simulink model "EKFSim"  (R2025b)
settings: Solver=FixedStepAuto  StartTime=0.0  StopTime=4500  RelTol=1e-3
values from neighbouring files (symbols this model uses):
  C1_bp = interp1(ECM.SOC_table, ECM.C1_table, SOC_bp, 'pchip')    [preparer_LUT_pour_EKFSim.m]
  OCV_bp = ppval(ECM.pp_OCV, SOC_bp)    [preparer_LUT_pour_EKFSim.m]
  R0_bp = interp1(ECM.SOC_table, ECM.R0_table, SOC_bp, 'pchip')    [preparer_LUT_pour_EKFSim.m]
  R1_bp = interp1(ECM.SOC_table, ECM.R1_table, SOC_bp, 'pchip')    [preparer_LUT_pour_EKFSim.m]
  SOC_bp = (5:1:100)' / 100    [preparer_LUT_pour_EKFSim.m]
libraries: fl_lib x7, nesl_utility x7
settings Model: Creator=WL  LastModifiedBy=SAT
settings SolverCC: AlgebraicLoopSolver=TrustRegion
settings DataIOCC: ReturnWorkspaceOutputs=off
settings DebuggingCC: UnconnectedInputMsg=warning  UnconnectedOutputMsg=warning  UnconnectedLineMsg=warning  ArithmeticOperatorsInVariantConditions=warning
settings ModelReferenceCC: EnableRefExpFcnMdlSchedulingChecks=on
settings SFSimCC: SimUseLocalCustomCode=off  CustomCodeUndefinedFunction=UseInterfaceOnly
settings RTWCC: GenCodeOnly=on  RTWUseLocalCustomCode=off  GPUComputeCapability=3.5
settings CodeAppCC: StateflowObjectComments=on

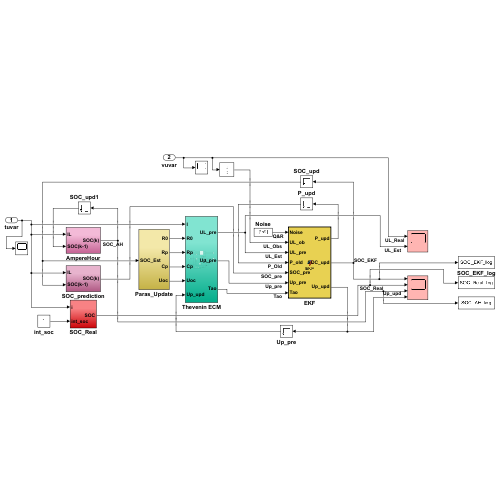
[thumbnail: Simulink's stored preview of the top-level diagram]
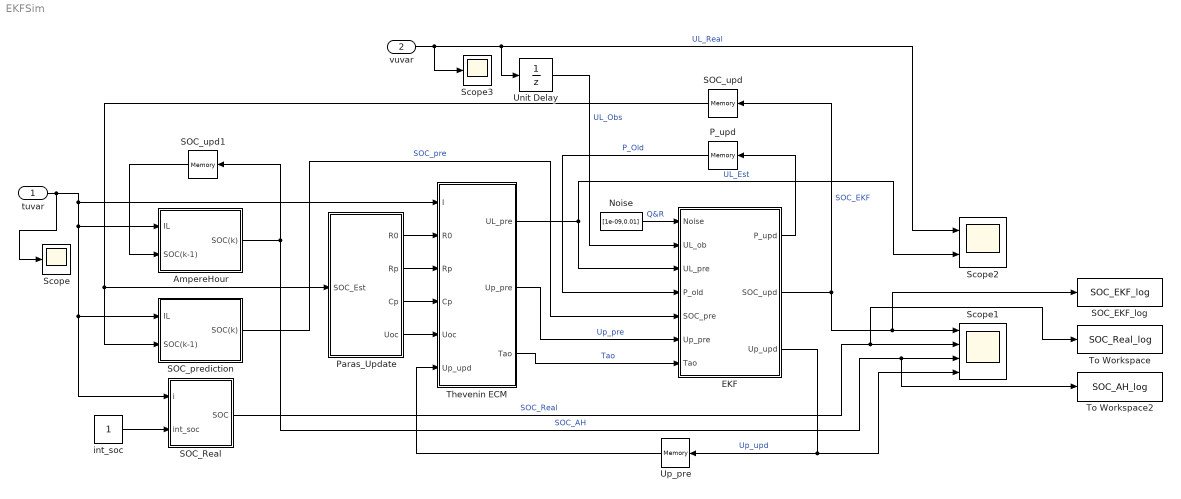
== system EKFSim ==
  tuvar : Inport  OutDataTypeStr=double
  vuvar : Inport  Port=2  OutDataTypeStr=double
  AmpereHour : Subsystem
  EKF : MATLAB Function  TreatAsAtomicUnit=on
  Noise : Constant  Value=[1e-09,0.01]
  P_upd : Memory  InitialCondition=[0.02 0 0 0.01]  InheritSampleTime=on  LinearizeAsDelay=on
  Paras_Update : Subsystem
  SOC_EKF_log : ToWorkspace  VariableName=SOC_EKF_log  SampleTime=-1
  SOC_Real : Subsystem
  SOC_prediction : Subsystem
  SOC_upd : Memory  InitialCondition=1  InheritSampleTime=on  LinearizeAsDelay=on
  SOC_upd1 : Memory  InitialCondition=1  InheritSampleTime=on  LinearizeAsDelay=on
  Scope : Scope
      settings: ActiveDisplayYMinimum=-18.981393680658311  ActiveDisplayYMaximum=11.78942945455692
  Scope1 : Scope  NumInputPorts=4
      settings: ActiveDisplayYMinimum=-0.2544970250554105  ActiveDisplayYMaximum=1.3066318096988883  DataLoggingVariableName=ScopeData2
  Scope2 : Scope  NumInputPorts=2
      settings: ActiveDisplayYMinimum=2.9853  ActiveDisplayYMaximum=4.38231  DataLoggingVariableName=ScopeData2
  Scope3 : Scope
      settings: ActiveDisplayYMinimum=-13.743145742790805  ActiveDisplayYMaximum=10.36659934742335  DataLoggingVariableName=ScopeData3
  Thevenin ECM : Subsystem
  To Workspace : ToWorkspace  VariableName=SOC_Real_log  SampleTime=-1
  To Workspace2 : ToWorkspace  VariableName=SOC_AH_log  SampleTime=-1
  Unit Delay : UnitDelay  InitialCondition=4.107  SampleTime=0.1  HasFrameUpgradeWarning=on
  Up_pre : Memory  InheritSampleTime=on  LinearizeAsDelay=on
  int_soc : Constant
  wires:
  Paras_Update/4(Uoc) -> Thevenin ECM/5(Uoc)
  Paras_Update/1(R0) -> Thevenin ECM/2(R0)
  int_soc/1 -> SOC_Real/2(int_soc)
  Paras_Update/3(Cp) -> Thevenin ECM/4(Cp)
  Paras_Update/2(Rp) -> Thevenin ECM/3(Rp)
  Thevenin ECM/1(UL_pre) -> Scope2/2, EKF/3(UL_pre)  "UL_Est"
  vuvar/1 -> Scope3/1, Unit Delay/1, Scope2/1  "UL_Real"
  SOC_Real/1(SOC) -> To Workspace/1, Scope1/2  "SOC_Real"
  Thevenin ECM/2(Up_pre) -> EKF/6(Up_pre)  "Up_pre"
  Noise/1 -> EKF/1(Noise)  "Q&R"
  SOC_prediction/1(SOC(k)) -> EKF/5(SOC_pre)  "SOC_pre"
  P_upd/1 -> EKF/4(P_old)  "P_Old"
  SOC_upd/1 -> SOC_prediction/2(SOC(k-1)), Paras_Update/1(SOC_Est)
  EKF/1(P_upd) -> P_upd/1
  Thevenin ECM/3(Tao) -> EKF/7(Tao)  "Tao"
  EKF/3(Up_upd) -> Scope1/4, Up_pre/1  "Up_upd"
  Up_pre/1 -> Thevenin ECM/6(Up_upd)
  EKF/2(SOC_upd) -> SOC_EKF_log/1, Scope1/1, SOC_upd/1  "SOC_EKF"
  Unit Delay/1 -> EKF/2(UL_ob)  "UL_Obs"
  AmpereHour/1(SOC(k)) -> To Workspace2/1, Scope1/3, SOC_upd1/1  "SOC_AH"
  tuvar/1 -> Scope/1, SOC_prediction/1(IL), SOC_Real/1(i), AmpereHour/1(IL), Thevenin ECM/1(I)
  SOC_upd1/1 -> AmpereHour/2(SOC(k-1))

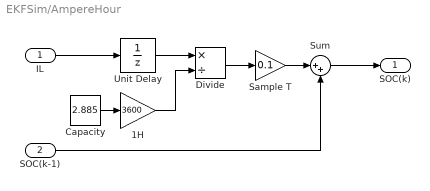
== system EKFSim/AmpereHour ==
  IL : Inport
  SOC(k-1) : Inport  Port=2
  1H : Gain  Gain=3600
  Capacity : Constant  Value=2.885
  Divide : Product  Inputs=*/
  Sample T : Gain  Gain=0.1
  Sum : Sum  Inputs=|++
  Unit Delay : UnitDelay  SampleTime=-1  HasFrameUpgradeWarning=on
  SOC(k) : Outport  VectorParamsAs1DForOutWhenUnconnected=off
  wires:
  Sample T/1 -> Sum/1
  Unit Delay/1 -> Divide/1
  SOC(k-1)/1 -> Sum/2
  IL/1 -> Unit Delay/1
  Sum/1 -> SOC(k)/1
  Capacity/1 -> 1H/1
  1H/1 -> Divide/2
  Divide/1 -> Sample T/1

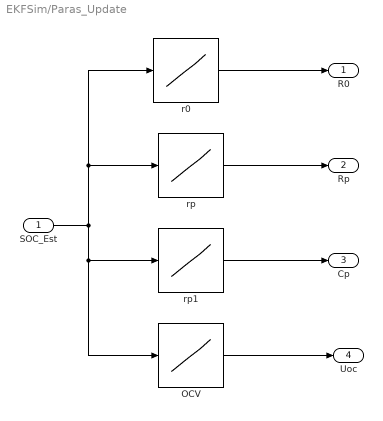
== system EKFSim/Paras_Update ==
  SOC_Est : Inport
  OCV : Lookup_n-D  NumberOfTableDimensions=1  BreakpointsForDimension1=SOC_bp  Table=OCV_bp  ExtrapMethod=Clip  InternalRulePriority=Speed  RndMeth=Simplest
  r0 : Lookup_n-D  NumberOfTableDimensions=1  BreakpointsForDimension1=SOC_bp  Table=R0_bp  ExtrapMethod=Clip  InternalRulePriority=Speed  RndMeth=Simplest
  rp : Lookup_n-D  NumberOfTableDimensions=1  BreakpointsForDimension1=SOC_bp  Table=R1_bp  ExtrapMethod=Clip  InternalRulePriority=Speed  RndMeth=Simplest
  rp1 : Lookup_n-D  NumberOfTableDimensions=1  BreakpointsForDimension1=SOC_bp  Table=C1_bp  ExtrapMethod=Clip  InternalRulePriority=Speed  RndMeth=Simplest
  R0 : Outport  VectorParamsAs1DForOutWhenUnconnected=off
  Rp : Outport  Port=2  VectorParamsAs1DForOutWhenUnconnected=off
  Cp : Outport  Port=3  VectorParamsAs1DForOutWhenUnconnected=off
  Uoc : Outport  Port=4  VectorParamsAs1DForOutWhenUnconnected=off
  wires:
  SOC_Est/1 -> OCV/1, rp1/1, rp/1, r0/1
  rp/1 -> Rp/1
  OCV/1 -> Uoc/1
  r0/1 -> R0/1
  rp1/1 -> Cp/1

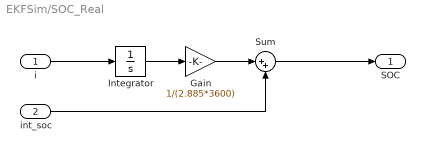
== system EKFSim/SOC_Real ==
  i : Inport
  int_soc : Inport  Port=2
  Gain : Gain  Gain=1/(2.885*3600)
  Integrator : Integrator
  Sum : Sum  Inputs=|++
  SOC : Outport  VectorParamsAs1DForOutWhenUnconnected=off
  wires:
  Gain/1 -> Sum/1
  Integrator/1 -> Gain/1
  int_soc/1 -> Sum/2
  i/1 -> Integrator/1
  Sum/1 -> SOC/1

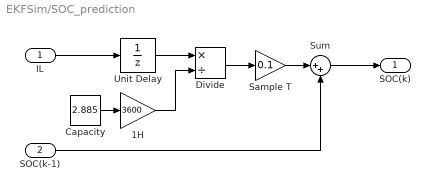
== system EKFSim/SOC_prediction ==
  IL : Inport
  SOC(k-1) : Inport  Port=2
  1H : Gain  Gain=3600
  Capacity : Constant  Value=2.885
  Divide : Product  Inputs=*/
  Sample T : Gain  Gain=0.1
  Sum : Sum  Inputs=|++
  Unit Delay : UnitDelay  SampleTime=-1  HasFrameUpgradeWarning=on
  SOC(k) : Outport  VectorParamsAs1DForOutWhenUnconnected=off
  wires:
  Sample T/1 -> Sum/1
  Unit Delay/1 -> Divide/1
  SOC(k-1)/1 -> Sum/2
  IL/1 -> Unit Delay/1
  Sum/1 -> SOC(k)/1
  Capacity/1 -> 1H/1
  1H/1 -> Divide/2
  Divide/1 -> Sample T/1

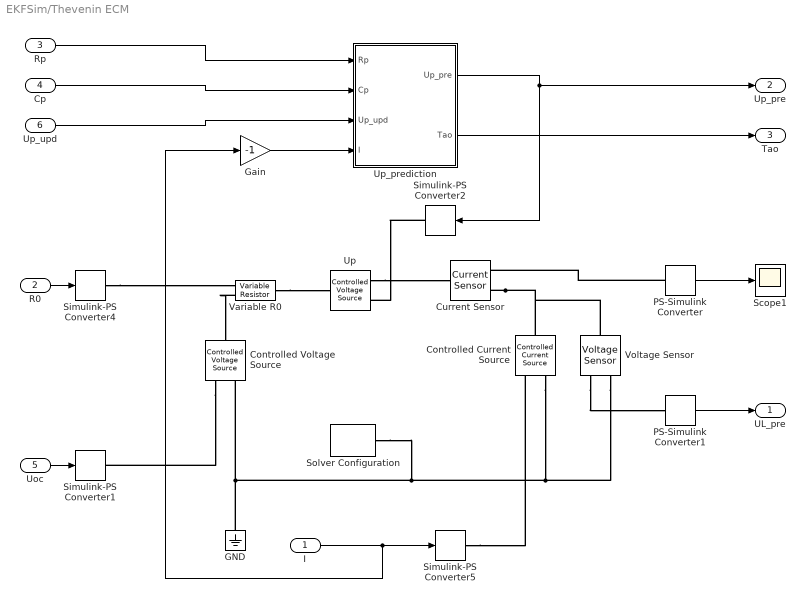
== system EKFSim/Thevenin ECM ==
  I : Inport
  R0 : Inport  Port=2
  Rp : Inport  Port=3
  Cp : Inport  Port=4
  Uoc : Inport  Port=5
  Up_upd : Inport  Port=6
  Controlled Current Source : fl_lib/Electrical/Electrical Sources/Controlled Current Source
  Controlled Voltage Source : fl_lib/Electrical/Electrical Sources/Controlled Voltage Source
  Current Sensor : fl_lib/Electrical/Electrical Sensors/Current Sensor
  GND : fl_lib/Electrical/Electrical Elements/Electrical Reference
  Gain : Gain  Gain=-1
  PS-Simulink Converter : nesl_utility/PS-Simulink Converter  PhysicalDomain=network_engine_domain  SubClassName=ps_output  LeftPortType=input  RightPortType=output  PseudoPeriodic=off  Frequencies=[]  VectorFormat=1-D array  Unit=A  AffineConversion=off
  PS-Simulink Converter1 : nesl_utility/PS-Simulink Converter  PhysicalDomain=network_engine_domain  SubClassName=ps_output  LeftPortType=input  RightPortType=output  PseudoPeriodic=off  Frequencies=[]  VectorFormat=1-D array  Unit=V  AffineConversion=off
  Scope1 : Scope
      settings: ActiveDisplayYMinimum=-63.1775  ActiveDisplayYMaximum=62.5975
  Simulink-PS Converter{1..2,4..5} (4 alike) : nesl_utility/Simulink-PS Converter  PhysicalDomain=network_engine_domain  SubClassName=ps_input  LeftPortType=input  RightPortType=output  PseudoPeriodic=off  Frequencies=[]  NoiseDistribution=none  NoiseParameters=[]  Unit=1  AffineConversion=off  FilteringAndDerivatives=zero  SimscapeFilterOrder=1  InputFilterTimeConstant=0.001  UdotUserProvided=0
  Solver Configuration : nesl_utility/Solver Configuration  PhysicalDomain=network_engine_domain  SubClassName=solver  LeftPortType=input  RightPortType=generic  Tones=[]  Harmonics=[]  SimulateNoise=off  Profile=off  UseLocalSampling=off  EnableSwitchedLinearOptims=on  FrequencyDomain=off  UseCCode=off  RelTol=0.001  AbsTol=1e-06  MinStep=1e-09  ToWorkspace=off  RevertToSquareIcSolve=off  NumHomotopyIterations=100  PhasorMode=off  PhasorModeNumHarmonics=1  ConsistencySolver=NEWTON_FTOL  IndexReductionMethod=DerivativeReplacement  DoDC=off  ResidualTolerance=1e-09  ConsistencyTolSource=GLOBAL  ConsistencyAbsTol=0.001  ConsistencyRelTol=0.001  ConsistencyTolFactor=0.001  UseLocalSolver=off  LocalSolverChoice=NE_BACKWARD_EULER_ADVANCER  ResolveIndetEquations=on  FunctionEvalNumThread=1  LocalSolverSampleTime=0.001  DoFixedCost=off  MaxNonlinIter=3  MaxModeIter=2  ComputeImpulses=off  ImpulseIterations=2  LinearAlgebra=Sparse  LinearAlgebraNumThread=0  EquationFormulation=NE_TIME_EF  DelaysMemoryBudget=1024  AutomaticFiltering=on  FilteringTimeConstant=0.001  PartitionStorageMethod=AS_NEEDED  PartitionMemoryBudget=1024  PartitionMethod=FAST  MultibodyUseLocalSolver=off  MultibodyLocalSolverChoice=ODE1  MultibodyLocalSolverSampleTime=0.001
  Up : fl_lib/Electrical/Electrical Sources/Controlled Voltage Source
  Up_prediction : MATLAB Function  TreatAsAtomicUnit=on
  Variable R0 : fl_lib/Electrical/Electrical Elements/Variable Resistor  Rmin=0 Ohm  thermalEnable=false  thermal_mass=1 J/K  i_specify=off  i_priority=None  i=0 A  i_nominal_specify=off  i_nominal_value=1  i_nominal_unit=A  v_specify=off  v_priority=None  v=0 V  v_nominal_specify=off  v_nominal_value=1  v_nominal_unit=V  T_specify=off  T_priority=None  T=300 K  T_nominal_specify=off  T_nominal_value=1  T_nominal_unit=K
  Voltage Sensor : fl_lib/Electrical/Electrical Sensors/Voltage Sensor
  UL_pre : Outport  VectorParamsAs1DForOutWhenUnconnected=off
  Up_pre : Outport  Port=2  VectorParamsAs1DForOutWhenUnconnected=off
  Tao : Outport  Port=3  VectorParamsAs1DForOutWhenUnconnected=off
  wires:
  PS-Simulink Converter1/1 -> UL_pre/1
  Uoc/1 -> Simulink-PS Converter1/1
  Cp/1 -> Up_prediction/2(Cp)
  Rp/1 -> Up_prediction/1(Rp)
  R0/1 -> Simulink-PS Converter4/1
  I/1 -> Gain/1, Simulink-PS Converter5/1
  PS-Simulink Converter/1 -> Scope1/1
  Up_prediction/1(Up_pre) -> Simulink-PS Converter2/1, Up_pre/1
  Up_upd/1 -> Up_prediction/3(Up_upd)
  Up_prediction/2(Tao) -> Tao/1
  Gain/1 -> Up_prediction/4(I)
  connections:
  Variable R0/LConn2 -- Controlled Voltage Source/LConn1
  Current Sensor/RConn2 -- Voltage Sensor/LConn1 -- Controlled Current Source/LConn1
  Voltage Sensor/RConn2 -- Controlled Current Source/RConn2 -- Solver Configuration/RConn1 -- Controlled Voltage Source/RConn2 -- GND/LConn1
  PS-Simulink Converter/LConn1 -- Current Sensor/RConn1
  Voltage Sensor/RConn1 -- PS-Simulink Converter1/LConn1
  Controlled Voltage Source/RConn1 -- Simulink-PS Converter1/RConn1
  Simulink-PS Converter5/RConn1 -- Controlled Current Source/RConn1
  Simulink-PS Converter4/RConn1 -- Variable R0/LConn1
  Variable R0/RConn1 -- Up/LConn1
  Up/RConn2 -- Current Sensor/LConn1
  Simulink-PS Converter2/RConn1 -- Up/RConn1

== matlab function EKFSim/Thevenin ECM/Up_prediction ==
  data: Rp input; Up_pre output; Cp input; Up_upd input; Tao output; I input
function [Up_pre, Tao] = fcn(Rp, Cp,Up_upd,I)
Ts = 0.1;
Tao = Rp*Cp;
Up_pre = exp(-Ts/Tao)*Up_upd + Rp*(1-exp(-Ts/Tao))*I;
end

== matlab function EKFSim/EKF ==
  data: P_upd output; Noise input; UL_ob input; UL_pre input; P_old input; SOC_pre input; Up_pre input; Tao input; SOC_upd output; Up_upd output
function [P_upd,SOC_upd,Up_upd] = EKF(Noise, UL_ob, UL_pre, P_old, SOC_pre, Up_pre, Tao)
Ts = 0.1;    % <-- MÊME Ts que dans Thevenin ECM
Q = Noise(1);
R = Noise(2);

A1 = 1;
A2 = exp(-Ts/Tao);
A = [A1 0;0 A2];

P_last = [P_old(1) P_old(2);P_old(3) P_old(4)];
P_pre = A*P_last*A' + [Q 0;0 Q];

SOC_vec  = [0.05 0.1 0.15 0.2 0.25 0.3 0.4 0.5 0.6 0.7 0.8 0.9 0.95 1];
dOCV_vec = [7.162 4.878 1.933 0.933 0.583 0.589667 0.6755 1.1175 1.1305 0.7665 0.933 1.135 1.401 1.642];
C1 = interp1(SOC_vec, dOCV_vec, SOC_pre, 'pchip', 'extrap');
C = [C1 -1];

X_pre = [SOC_pre;Up_pre];
K = P_pre*C'*(C*P_pre*C'+ R)^(-1);
X_upd = X_pre + K*(UL_ob-UL_pre);
P_update = P_pre - K*C*P_pre;

SOC_upd = X_upd(1);
Up_upd = X_upd(2);
P_upd = [P_update(1,1) P_update(1,2) P_update(2,1) P_update(2,2)];
end
